simulink subsystem "Model_of_Actuators"  (R2025b)
settings: Solver=VariableStepAuto  StartTime=0.0  StopTime=10.0  RelTol=1e-3
settings Model: Creator=Admin  LastModifiedBy=Admin

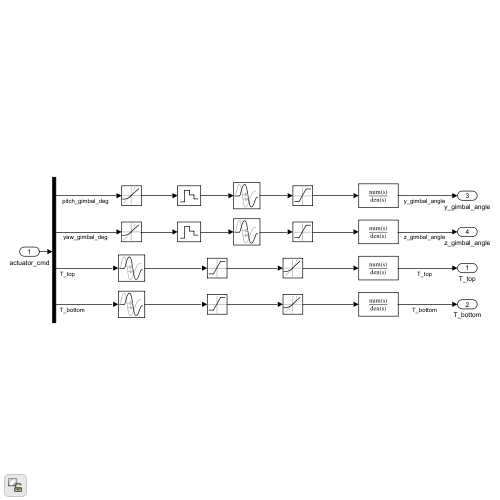
[thumbnail: Simulink's stored preview of the top-level diagram]
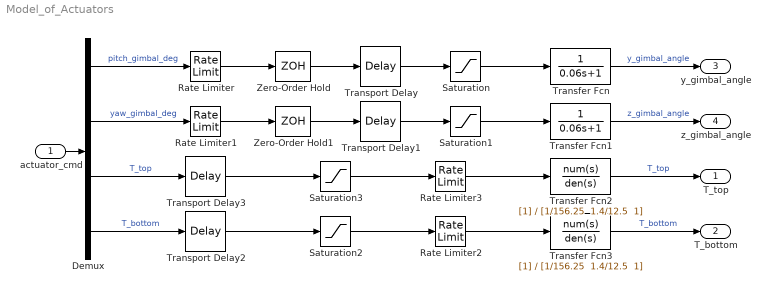
== system Model_of_Actuators ==
  actuator_cmd : Inport
  Demux : Demux
  Rate Limiter : RateLimiter  RisingSlewLimit=300  FallingSlewLimit=-300  SampleTimeMode=inherited
  Rate Limiter1 : RateLimiter  RisingSlewLimit=300  FallingSlewLimit=-300  SampleTimeMode=inherited
  Rate Limiter2 : RateLimiter  RisingSlewLimit=300  FallingSlewLimit=-500  SampleTimeMode=inherited
  Rate Limiter3 : RateLimiter  RisingSlewLimit=300  FallingSlewLimit=-500  SampleTimeMode=inherited
  Saturation : Saturate  UpperLimit=15  LowerLimit=-15
  Saturation1 : Saturate  UpperLimit=15  LowerLimit=-15
  Saturation2 : Saturate  UpperLimit=100  LowerLimit=0
  Saturation3 : Saturate  UpperLimit=100  LowerLimit=0
  Transfer Fcn : TransferFcn  Denominator=[0.06 1]
  Transfer Fcn1 : TransferFcn  Denominator=[0.06 1]
  Transfer Fcn2 : TransferFcn  Denominator="[1/156.25  1.4/12.5  1]"
  Transfer Fcn3 : TransferFcn  Denominator="[1/156.25  1.4/12.5  1]"
  Transport Delay : TransportDelay  DelayTime=0.02
  Transport Delay1 : TransportDelay  DelayTime=0.02
  Transport Delay2 : TransportDelay  DelayTime=0.1
  Transport Delay3 : TransportDelay  DelayTime=0.1
  Zero-Order Hold : ZeroOrderHold  SampleTime=0.02
  Zero-Order Hold1 : ZeroOrderHold  SampleTime=0.02
  T_top : Outport
  T_bottom : Outport  Port=2
  y_gimbal_angle : Outport  Port=3
  z_gimbal_angle : Outport  Port=4
  wires:
  Rate Limiter2/1 -> Transfer Fcn3/1
  Rate Limiter3/1 -> Transfer Fcn2/1
  Demux/2 -> Rate Limiter1/1  "yaw_gimbal_deg"
  Saturation/1 -> Transfer Fcn/1
  Saturation3/1 -> Rate Limiter3/1
  Rate Limiter1/1 -> Zero-Order Hold1/1
  Zero-Order Hold/1 -> Transport Delay/1
  Rate Limiter/1 -> Zero-Order Hold/1
  Saturation2/1 -> Rate Limiter2/1
  Transport Delay1/1 -> Saturation1/1
  Saturation1/1 -> Transfer Fcn1/1
  Zero-Order Hold1/1 -> Transport Delay1/1
  Transport Delay/1 -> Saturation/1
  Demux/1 -> Rate Limiter/1  "pitch_gimbal_deg"
  actuator_cmd/1 -> Demux/1
  Transfer Fcn2/1 -> T_top/1  "T_top"
  Transfer Fcn3/1 -> T_bottom/1  "T_bottom"
  Transfer Fcn/1 -> y_gimbal_angle/1  "y_gimbal_angle"
  Transfer Fcn1/1 -> z_gimbal_angle/1  "z_gimbal_angle"
  Demux/3 -> Transport Delay3/1  "T_top"
  Transport Delay3/1 -> Saturation3/1
  Demux/4 -> Transport Delay2/1  "T_bottom"
  Transport Delay2/1 -> Saturation2/1
